simulink model "mpc_psm"  (R2026b)
settings: Solver=ode23tb  StopTime=param.sim.simlength  FixedStep=param.glb_time.tc  MaxStep=param.glb_time.tc
values from neighbouring files (symbols this model uses):
  param = struct()    [init_model.m]
undefined symbols (not defined in the file or in its folder): tc
libraries: fl_lib x28, nesl_utility x13, cstblocks_lti x6, lithium_ion_battery x1, dclink_with_center_tap x1, ideal_bridges_lib x1, dead_time_generator_cmos_simulink x1, single_phase_pwm_modulator x1, threephase_inductor_lib x1, simple_flexible_shaft x1, permanent_magnet_synchronous_machine x1
(part 2 of 3)

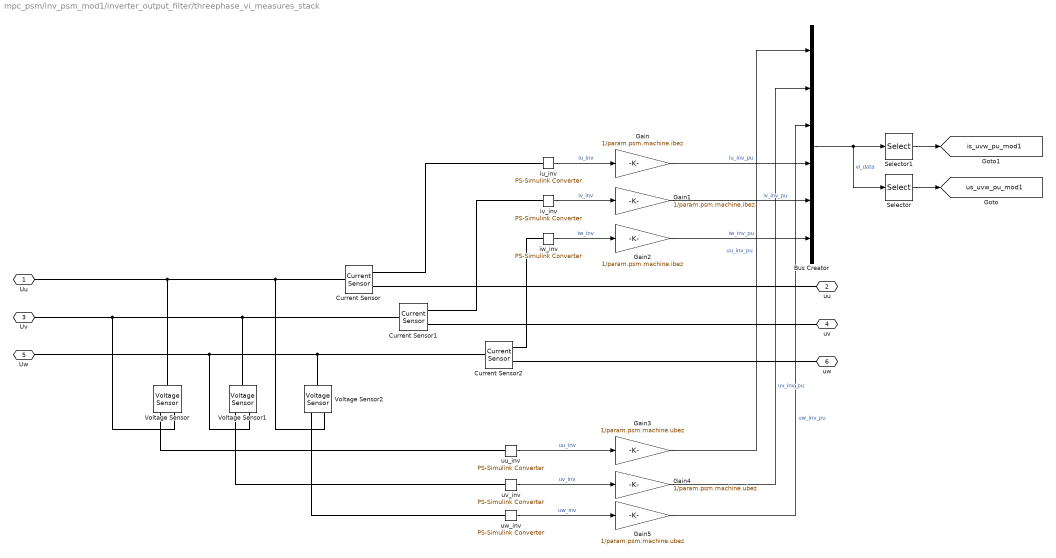
== system mpc_psm/inv_psm_mod1/inverter_output_filter/threephase_vi_measures_stack ==
  Bus Creator : BusCreator  Inputs=6
  Current Sensor : fl_lib/Electrical/Electrical Sensors/Current Sensor
  Current Sensor1 : fl_lib/Electrical/Electrical Sensors/Current Sensor
  Current Sensor2 : fl_lib/Electrical/Electrical Sensors/Current Sensor
  Gain : Gain  Gain=1/param.psm.machine.ibez
  Gain1 : Gain  Gain=1/param.psm.machine.ibez
  Gain2 : Gain  Gain=1/param.psm.machine.ibez
  Gain3 : Gain  Gain=1/param.psm.machine.ubez
  Gain4 : Gain  Gain=1/param.psm.machine.ubez
  Gain5 : Gain  Gain=1/param.psm.machine.ubez
  Selector : Selector  InputPortWidth=6  IndexOptions=Index vector (dialog)  Indices=[1 2 3]  OutputSizes=1  RuntimeRangeChecks=off
  Selector1 : Selector  InputPortWidth=6  IndexOptions=Index vector (dialog)  Indices=[4 5 6]  OutputSizes=1  RuntimeRangeChecks=off
  Voltage Sensor : fl_lib/Electrical/Electrical Sensors/Voltage Sensor
  Voltage Sensor1 : fl_lib/Electrical/Electrical Sensors/Voltage Sensor
  Voltage Sensor2 : fl_lib/Electrical/Electrical Sensors/Voltage Sensor
  iu_inv : nesl_utility/PS-Simulink Converter  PhysicalDomain=network_engine_domain  SubClassName=ps_output  LeftPortType=input  RightPortType=output  PseudoPeriodic=off  Frequencies=[]  VectorFormat=1-D array  Unit=A  AffineConversion=off
  iv_inv : nesl_utility/PS-Simulink Converter  PhysicalDomain=network_engine_domain  SubClassName=ps_output  LeftPortType=input  RightPortType=output  PseudoPeriodic=off  Frequencies=[]  VectorFormat=1-D array  Unit=A  AffineConversion=off
  iw_inv : nesl_utility/PS-Simulink Converter  PhysicalDomain=network_engine_domain  SubClassName=ps_output  LeftPortType=input  RightPortType=output  PseudoPeriodic=off  Frequencies=[]  VectorFormat=1-D array  Unit=A  AffineConversion=off
  uu_inv : nesl_utility/PS-Simulink Converter  PhysicalDomain=network_engine_domain  SubClassName=ps_output  LeftPortType=input  RightPortType=output  PseudoPeriodic=off  Frequencies=[]  VectorFormat=1-D array  Unit=V  AffineConversion=off
  uv_inv : nesl_utility/PS-Simulink Converter  PhysicalDomain=network_engine_domain  SubClassName=ps_output  LeftPortType=input  RightPortType=output  PseudoPeriodic=off  Frequencies=[]  VectorFormat=1-D array  Unit=V  AffineConversion=off
  uw_inv : nesl_utility/PS-Simulink Converter  PhysicalDomain=network_engine_domain  SubClassName=ps_output  LeftPortType=input  RightPortType=output  PseudoPeriodic=off  Frequencies=[]  VectorFormat=1-D array  Unit=V  AffineConversion=off
  Uu : PMIOPort  Side=Left
  uu : PMIOPort  Port=2  Side=Right
  Uv : PMIOPort  Port=3  Side=Left
  uv : PMIOPort  Port=4  Side=Right
  Uw : PMIOPort  Port=5  Side=Left
  uw : PMIOPort  Port=6  Side=Right
  tag scope: is_uvw_pu_mod1=global, us_uvw_pu_mod1=global
  wires:
  Bus Creator/1 -> Selector/1, Selector1/1  "vi_data"
  Selector/1 -> [us_uvw_pu_mod1]
  iv_inv/1 -> Gain1/1  "iv_inv"
  iu_inv/1 -> Gain/1  "iu_inv"
  iw_inv/1 -> Gain2/1  "iw_inv"
  uu_inv/1 -> Gain3/1  "uu_inv"
  uv_inv/1 -> Gain4/1  "uv_inv"
  uw_inv/1 -> Gain5/1  "uw_inv"
  Selector1/1 -> [is_uvw_pu_mod1]
  Gain/1 -> Bus Creator/4  "iu_inv_pu"
  Gain1/1 -> Bus Creator/5  "iv_inv_pu"
  Gain2/1 -> Bus Creator/6  "iw_inv_pu"
  Gain3/1 -> Bus Creator/1  "uu_inv_pu"
  Gain4/1 -> Bus Creator/2  "uv_inv_pu"
  Gain5/1 -> Bus Creator/3  "uw_inv_pu"
  connections:
  Current Sensor1/LConn1 -- Voltage Sensor1/LConn1 -- Voltage Sensor/RConn2 -- Uv/RConn1
  Voltage Sensor/RConn1 -- uu_inv/LConn1
  Current Sensor/RConn2 -- uu/RConn1
  Voltage Sensor1/RConn1 -- uv_inv/LConn1
  Voltage Sensor2/LConn1 -- Current Sensor2/LConn1 -- Voltage Sensor1/RConn2 -- Uw/RConn1
  Current Sensor/LConn1 -- Voltage Sensor2/RConn2 -- Uu/RConn1 -- Voltage Sensor/LConn1
  Current Sensor1/RConn2 -- uv/RConn1
  Voltage Sensor2/RConn1 -- uw_inv/LConn1
  iv_inv/LConn1 -- Current Sensor1/RConn1
  iu_inv/LConn1 -- Current Sensor/RConn1
  iw_inv/LConn1 -- Current Sensor2/RConn1
  Current Sensor2/RConn2 -- uw/RConn1

== system mpc_psm/inv_psm_mod1/inverter/inverter/timer ==
  time_source : Inport
  Constant1 : Constant  Value=double_sampling
  Constant2 : Constant  Value=0
  Constant8 : Constant  Value=tc
  Constant9 : Constant  Value=f
  MATLAB Function : MATLAB Function  TreatAsAtomicUnit=on  SystemSampleTime=tc
  MATLAB Function1 : single_phase_pwm_modulator/Single phase two level PWM generator with global TRGO/MATLAB Function1  SystemSampleTime=tc  VariantActivationTime=update diagram  EmptyChoice=off  PassThrough=off  PassThroughVariantControl=(default)  EmptyChoiceVariantControl=(default)  AllowFlexibleInterface=on  Latency=0  AutoFrameSizeCalculation=off
  period : Constant  Value=1/f
  TRGO : Outport
  wires:
  Constant1/1 -> MATLAB Function1/4
  time_source/1 -> MATLAB Function/1(t)
  Constant9/1 -> MATLAB Function1/2
  Constant8/1 -> MATLAB Function1/1
  MATLAB Function1/1 -> TRGO/1
  MATLAB Function/1(y) -> MATLAB Function1/3
  Constant2/1 -> MATLAB Function/2(phase)
  period/1 -> MATLAB Function/3(period)

== system mpc_psm/inv_psm_mod1/inverter_ctrl/inverter_control/Speed control ==
  rotor speed : Inport
  rotor speed ref : Inport  Port=2
  1/Ti : Gain  Gain=param.psm.ctrl.kp_w  SaturateOnIntegerOverflow=on  OutDataTypeStr=Inherit: Same as input  ParamDataTypeStr=Inherit: Same as input
  Saturation : Saturate  UpperLimit=param.psm.ctrl.iq_lim  LowerLimit=-param.psm.ctrl.iq_lim
  Sum1 : Sum  Inputs=+++  SaturateOnIntegerOverflow=on
  Sum2 : Sum  Inputs=-+  SaturateOnIntegerOverflow=on
  Sum3 : Sum  Inputs=-+  SaturateOnIntegerOverflow=on
  Unit Delay4 : UnitDelay  SampleTime=-1
  kp : Gain  Gain=param.psm.ctrl.ki_w*param.glb_time.ts_inv  SaturateOnIntegerOverflow=on  OutDataTypeStr=Inherit: Same as input  ParamDataTypeStr=Inherit: Same as input
  torque_ref : Outport
  wires:
  1/Ti/1 -> Sum1/1, Sum3/1
  kp/1 -> Sum1/2
  Sum3/1 -> Unit Delay4/1
  Unit Delay4/1 -> Sum1/3
  rotor speed ref/1 -> Sum2/2
  rotor speed/1 -> Sum2/1
  Sum2/1 -> kp/1, 1/Ti/1
  Sum1/1 -> Saturation/1
  Saturation/1 -> Sum3/2, torque_ref/1

== system mpc_psm/inv_psm_mod1/inverter_ctrl/inverter_control/encoder-sensorless-switch ==
  Constant : Constant  Value=param.psm.ctrl.omega_th
  MATLAB Function : MATLAB Function  TreatAsAtomicUnit=on
  Variant Source1 : VariantSource  VariantControls={param.psm.mode.use_psm_encoder == 1, param.psm.mode.use_psm_encoder == 0}
  Variant Source2 : VariantSource  VariantControls={param.psm.mode.use_psm_encoder == 1, param.psm.mode.use_psm_encoder == 0}
  double_integrator_observer : Subsystem
  omega_pu_psm/hat1 : Scope  NumInputPorts=2
      settings: ActiveDisplayYMinimum=0.7763345893279654  ActiveDisplayYMaximum=1.2909010705406665  DataLoggingVariableName=ScopeData13
  theta_elec_psm/hat : Scope  NumInputPorts=2
      settings: ActiveDisplayYMinimum=-1  ActiveDisplayYMaximum=1  DataLoggingVariableName=ScopeData12
  tag scope: motor_phase_ctrl_mod1=scoped, motor_speed_pu_ctrl_mod1=scoped
  wires:
  Variant Source1/1 -> [motor_speed_pu_ctrl_mod1]
  Variant Source2/1 -> [motor_phase_ctrl_mod1]
  [phase_hat_mod1] -> theta_elec_psm/hat/1  "theta_hat_mod1"
  [omega_hat_pu_mod1] -> omega_pu_psm/hat1/1  "omega_hat_pu_mod1"
  [phased_psm] -> double_integrator_observer/1(phase_psm)
  double_integrator_observer/1(omega_pu_psm_hat) -> MATLAB Function/1(omega_psm), Variant Source1/1, omega_pu_psm/hat1/2  "omega_pu_psm_hat"
  double_integrator_observer/2(phase_psm_hat) -> theta_elec_psm/hat/2, Variant Source2/1, MATLAB Function/2(phase_psm)  "theta_psm_hat"
  MATLAB Function/1(omega_ctrl) -> Variant Source1/2
  MATLAB Function/2(phase_ctrl) -> Variant Source2/2
  [omega_hat_pu_mod1] -> MATLAB Function/3(omega_obs)  "omega_hat_pu_mod1"
  [phase_hat_mod1] -> MATLAB Function/4(phase_obs)  "theta_hat_mod1"
  Constant/1 -> MATLAB Function/5(omega_th)

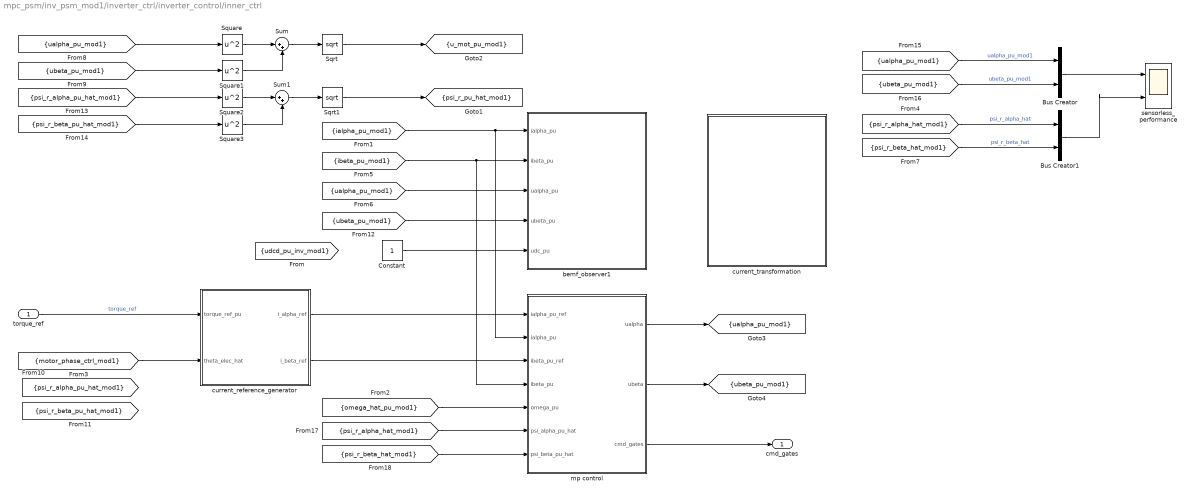
== system mpc_psm/inv_psm_mod1/inverter_ctrl/inverter_control/inner_ctrl ==
  torque_ref : Inport
  Bus Creator : BusCreator  Inputs=2
  Bus Creator1 : BusCreator  Inputs=2
  Constant : Constant
  Sqrt : Sqrt
  Sqrt1 : Sqrt
  Square{,1..3} (4 alike) : Math  Operator=square
  Sum : Sum  Inputs=|++
  Sum1 : Sum  Inputs=|++
  bemf_observer1 : Subsystem
  current_reference_generator : Subsystem
  current_transformation : Subsystem
  mp control : Subsystem
  sensorless_performance : Scope  NumInputPorts=2
      settings: ActiveDisplayYMinimum=-1.21322413533926  ActiveDisplayYMaximum=1.2041211351752281  DataLoggingVariableName=ScopeData5
  cmd_gates : Outport  VectorParamsAs1DForOutWhenUnconnected=off
  tag scope: psi_r_pu_hat_mod1=scoped, u_mot_pu_mod1=scoped, ualpha_pu_mod1=scoped, ubeta_pu_mod1=scoped
  wires:
  torque_ref/1 -> current_reference_generator/1(torque_ref_pu)  "torque_ref"
  [ibeta_pu_mod1] -> bemf_observer1/2(ibeta_pu), mp control/4(ibeta_pu)
  [ialpha_pu_mod1] -> bemf_observer1/1(ialpha_pu), mp control/2(ialpha_pu)
  [ualpha_pu_mod1] -> bemf_observer1/3(ualpha_pu)
  [ubeta_pu_mod1] -> bemf_observer1/4(ubeta_pu)
  Constant/1 -> bemf_observer1/5(udc_pu)
  [motor_phase_ctrl_mod1] -> current_reference_generator/2(theta_elec_hat)
  mp control/1(ualpha) -> [ualpha_pu_mod1]
  mp control/2(ubeta) -> [ubeta_pu_mod1]
  current_reference_generator/1(i_alpha_ref) -> mp control/1(ialpha_pu_ref)
  current_reference_generator/2(i_beta_ref) -> mp control/3(ibeta_pu_ref)
  [omega_hat_pu_mod1] -> mp control/5(omega_pu)
  [psi_r_alpha_hat_mod1] -> mp control/6(psi_alpha_pu_hat)
  [psi_r_beta_hat_mod1] -> mp control/7(psi_beta_pu_hat)
  mp control/3(cmd_gates) -> cmd_gates/1
  [ualpha_pu_mod1] -> Square/1
  [ubeta_pu_mod1] -> Square1/1
  Square/1 -> Sum/1
  Square1/1 -> Sum/2
  Sum/1 -> Sqrt/1
  Sqrt/1 -> [u_mot_pu_mod1]
  Sqrt1/1 -> [psi_r_pu_hat_mod1]
  Sum1/1 -> Sqrt1/1
  Square3/1 -> Sum1/2
  Square2/1 -> Sum1/1
  [psi_r_beta_pu_hat_mod1] -> Square3/1
  [psi_r_alpha_pu_hat_mod1] -> Square2/1
  [ualpha_pu_mod1] -> Bus Creator/1  "ualpha_pu_mod1"
  [ubeta_pu_mod1] -> Bus Creator/2  "ubeta_pu_mod1"
  [psi_r_beta_hat_mod1] -> Bus Creator1/2  "psi_r_beta_hat"
  [psi_r_alpha_hat_mod1] -> Bus Creator1/1  "psi_r_alpha_hat"
  Bus Creator/1 -> sensorless_performance/1
  Bus Creator1/1 -> sensorless_performance/2

== system mpc_psm/inv_psm_mod1/inverter_ctrl/inverter_control/is inv quantizzation and one step delay ==
  is_abc_pu : Inport
  Demux : Demux  Outputs=3
  Mux : Mux  Inputs=3
  is inv quantizzation and one step delay : Subsystem
  isd_abc_pu : Outport
  wires:
  is inv quantizzation and one step delay/2(isd_v_pu) -> Mux/2
  is_abc_pu/1 -> Demux/1
  is inv quantizzation and one step delay/3(isd_w_pu) -> Mux/3
  is inv quantizzation and one step delay/1(isd_u_pu) -> Mux/1
  Demux/1 -> is inv quantizzation and one step delay/1(is_u_pu)
  Mux/1 -> isd_abc_pu/1
  Demux/3 -> is inv quantizzation and one step delay/3(is_w_pu)
  Demux/2 -> is inv quantizzation and one step delay/2(is_v_pu)

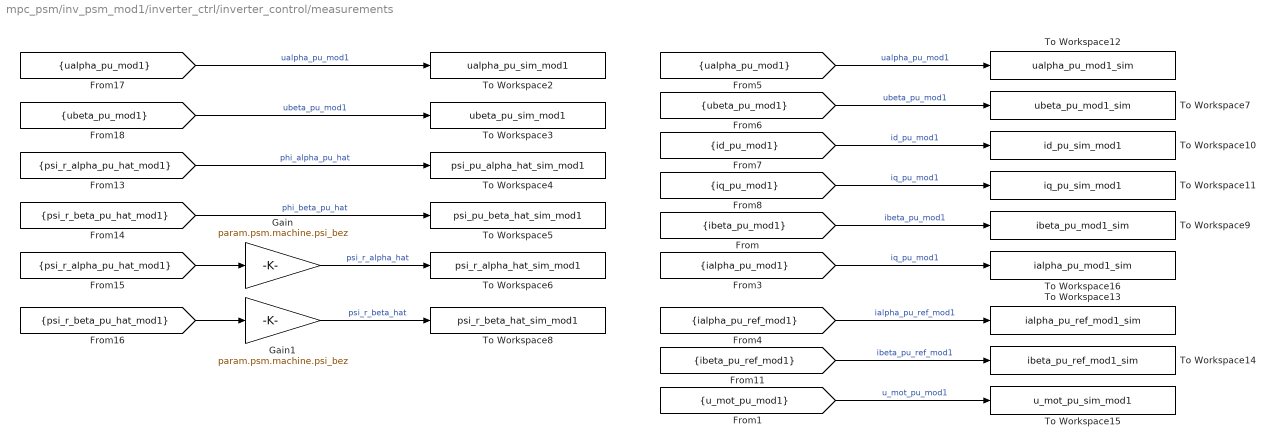
== system mpc_psm/inv_psm_mod1/inverter_ctrl/inverter_control/measurements ==
  Gain : Gain  Gain=param.psm.machine.psi_bez
  Gain1 : Gain  Gain=param.psm.machine.psi_bez
  To Workspace10 : ToWorkspace  VariableName=id_pu_sim_mod1  SampleTime=-1
      settings: MaxDataPoints=param.glb_time.Ns_inv
  To Workspace11 : ToWorkspace  VariableName=iq_pu_sim_mod1  SampleTime=-1
      settings: MaxDataPoints=param.glb_time.Ns_inv
  To Workspace12 : ToWorkspace  VariableName=ualpha_pu_mod1_sim  SampleTime=-1
      settings: MaxDataPoints=param.glb_time.Ns_inv
  To Workspace13 : ToWorkspace  VariableName=ialpha_pu_ref_mod1_sim  SampleTime=-1
      settings: MaxDataPoints=param.glb_time.Ns_inv
  To Workspace14 : ToWorkspace  VariableName=ibeta_pu_ref_mod1_sim  SampleTime=-1
      settings: MaxDataPoints=param.glb_time.Ns_inv
  To Workspace15 : ToWorkspace  VariableName=u_mot_pu_sim_mod1  SampleTime=-1
      settings: MaxDataPoints=param.glb_time.Ns_inv
  To Workspace16 : ToWorkspace  VariableName=ialpha_pu_mod1_sim  SampleTime=-1
      settings: MaxDataPoints=param.glb_time.Ns_inv
  To Workspace2 : ToWorkspace  VariableName=ualpha_pu_sim_mod1  SampleTime=-1
      settings: MaxDataPoints=param.glb_time.Ns_inv
  To Workspace3 : ToWorkspace  VariableName=ubeta_pu_sim_mod1  SampleTime=-1
      settings: MaxDataPoints=param.glb_time.Ns_inv
  To Workspace4 : ToWorkspace  VariableName=psi_pu_alpha_hat_sim_mod1  SampleTime=-1
      settings: MaxDataPoints=param.glb_time.Ns_inv
  To Workspace5 : ToWorkspace  VariableName=psi_pu_beta_hat_sim_mod1  SampleTime=-1
      settings: MaxDataPoints=param.glb_time.Ns_inv
  To Workspace6 : ToWorkspace  VariableName=psi_r_alpha_hat_sim_mod1  SampleTime=-1
      settings: MaxDataPoints=param.glb_time.Ns_inv
  To Workspace7 : ToWorkspace  VariableName=ubeta_pu_mod1_sim  SampleTime=-1
      settings: MaxDataPoints=param.glb_time.Ns_inv
  To Workspace8 : ToWorkspace  VariableName=psi_r_beta_hat_sim_mod1  SampleTime=-1
      settings: MaxDataPoints=param.glb_time.Ns_inv
  To Workspace9 : ToWorkspace  VariableName=ibeta_pu_mod1_sim  SampleTime=-1
      settings: MaxDataPoints=param.glb_time.Ns_inv
  wires:
  [psi_r_alpha_pu_hat_mod1] -> Gain/1
  [ualpha_pu_mod1] -> To Workspace2/1  "ualpha_pu_mod1"
  Gain/1 -> To Workspace6/1  "psi_r_alpha_hat"
  [psi_r_alpha_pu_hat_mod1] -> To Workspace4/1  "phi_alpha_pu_hat"
  [ubeta_pu_mod1] -> To Workspace3/1  "ubeta_pu_mod1"
  [psi_r_beta_pu_hat_mod1] -> To Workspace5/1  "phi_beta_pu_hat"
  Gain1/1 -> To Workspace8/1  "psi_r_beta_hat"
  [psi_r_beta_pu_hat_mod1] -> Gain1/1
  [u_mot_pu_mod1] -> To Workspace15/1  "u_mot_pu_mod1"
  [ialpha_pu_ref_mod1] -> To Workspace13/1  "ialpha_pu_ref_mod1"
  [ubeta_pu_mod1] -> To Workspace7/1  "ubeta_pu_mod1"
  [ualpha_pu_mod1] -> To Workspace12/1  "ualpha_pu_mod1"
  [iq_pu_mod1] -> To Workspace11/1  "iq_pu_mod1"
  [id_pu_mod1] -> To Workspace10/1  "id_pu_mod1"
  [ibeta_pu_ref_mod1] -> To Workspace14/1  "ibeta_pu_ref_mod1"
  [ibeta_pu_mod1] -> To Workspace9/1  "ibeta_pu_mod1"
  [ialpha_pu_mod1] -> To Workspace16/1  "iq_pu_mod1"

== system mpc_psm/inv_psm_mod1/inverter_ctrl/inverter_control/omega_acquisition ==
  omega_psm : Inport
  Gain : Gain  Gain=1/param.psm.machine.omega_bez
  Quantizer : Quantizer  QuantizationInterval=param.meas.adc_quantization
  Unit Delay : UnitDelay  SampleTime=-1
  Zero-Order Hold : ZeroOrderHold  SampleTime=-1
  omega_pu_psm : Outport
  wires:
  Quantizer/1 -> Unit Delay/1
  omega_psm/1 -> Gain/1
  Unit Delay/1 -> omega_pu_psm/1
  Zero-Order Hold/1 -> Quantizer/1
  Gain/1 -> Zero-Order Hold/1

== system mpc_psm/inv_psm_mod1/inverter_ctrl/inverter_control/omega_pu ==
  Abs : Abs  SaturateOnIntegerOverflow=off
  flt : Subsystem
  abs(omega_pu) : Outport
  omega_pu : Outport  Port=2
  wires:
  Abs/1 -> flt/1(input)
  [motor_speed_pu_ctrl_mod1] -> Abs/1, omega_pu/1
  flt/1(output) -> abs(omega_pu)/1

== system mpc_psm/inv_psm_mod1/inverter_ctrl/inverter_control/phase_acquisition ==
  phase_psm : Inport
  Quantizer : Quantizer  QuantizationInterval=param.meas.adc_quantization
  Unit Delay : UnitDelay  SampleTime=-1
  Zero-Order Hold : ZeroOrderHold  SampleTime=-1
  phased_psm : Outport
  wires:
  Zero-Order Hold/1 -> Quantizer/1
  Unit Delay/1 -> phased_psm/1
  phase_psm/1 -> Zero-Order Hold/1
  Quantizer/1 -> Unit Delay/1

== system mpc_psm/inv_psm_mod1/inverter_ctrl/inverter_control/phase_compensation_1 ==
  local_time : Inport
  master_time : Inport  Port=2
  Zero-Order Hold : ZeroOrderHold  SampleTime=-1
  Zero-Order Hold1 : ZeroOrderHold  SampleTime=-1
  alignment_ctrl : Subsystem
  y : Outport
  wires:
  local_time/1 -> Zero-Order Hold/1
  master_time/1 -> Zero-Order Hold1/1
  alignment_ctrl/1(dp) -> y/1
  Zero-Order Hold/1 -> alignment_ctrl/1(local_time)
  Zero-Order Hold1/1 -> alignment_ctrl/2(master_time)

== system mpc_psm/inv_psm_mod1/inverter_ctrl/inverter_control/speed_reference_generator ==
  Step : Step  Time=param.psm.mode.time_start_motor_control  FinalValue=param.load.omega_m_sim/param.psm.machine.omega_m_bez
  Step1 : Step  Commented=on  Time=param.sim.simlength/2  FinalValue=-2*param.load.omega_m_sim/param.psm.machine.omega_m_bez
  Sum : Sum  Inputs=|++
  flt : Subsystem
  omega_ref_pu : Outport
  tag scope: omega_ref_pu_mod1=global
  wires:
  Step/1 -> Sum/1
  Step1/1 -> Sum/2
  Sum/1 -> flt/1(input)
  flt/1(output) -> [omega_ref_pu_mod1], omega_ref_pu/1

== system mpc_psm/inv_psm_mod1/inverter_ctrl/inverter_control/torque_reference ==
  rotor speed : Inport
  1-D Lookup Table : Lookup_n-D  NumberOfTableDimensions=1  BreakpointsForDimension1=param.load.rpm_base  Table=param.load.torque_base  InternalRulePriority=Speed  RndMeth=Simplest
  Gain : Gain  Gain=param.load.torque_overload_factor
  Gain1 : Gain  Gain=1/param.psm.machine.tau_bez
  Gain2 : Gain  Gain=param.psm.machine.rpm_nom
  Gain3 : Gain  Gain=-1
  Saturation : Saturate  UpperLimit=0  LowerLimit=-inf
  torque_ref : Outport
  wires:
  rotor speed/1 -> Gain2/1
  Gain/1 -> Saturation/1
  Saturation/1 -> torque_ref/1
  Gain1/1 -> Gain3/1
  1-D Lookup Table/1 -> Gain1/1
  Gain2/1 -> 1-D Lookup Table/1
  Gain3/1 -> Gain/1

== system mpc_psm/inv_psm_mod1/inverter_ctrl/inverter_control/udc_acquisition ==
  udc_pu : Inport
  Quantizer : Quantizer  QuantizationInterval=param.meas.adc_quantization
  Unit Delay : UnitDelay  SampleTime=-1
  Zero-Order Hold : ZeroOrderHold  SampleTime=-1
  udcd_pu : Outport
  wires:
  Quantizer/1 -> Unit Delay/1
  udc_pu/1 -> Zero-Order Hold/1
  Unit Delay/1 -> udcd_pu/1
  Zero-Order Hold/1 -> Quantizer/1

== system mpc_psm/inv_psm_mod1/inverter_ctrl/inverter_control/encoder-sensorless-switch/double_integrator_observer ==
  phase_psm : Inport
  Dead Zone : DeadZone  LowerValue=-0.01  UpperValue=0.01
  Gain : Gain  Gain=param.psm.ctrl.di_obs.komega
  Gain1 : Gain  Gain=param.psm.ctrl.di_obs.ktheta
  Gain2 : Gain  Gain=param.psm.ctrl.omega_base
  Gain3 : Gain  Gain=1/param.psm.ctrl.omega_base
  Gain4 : Gain  Gain=param.glb_time.ts_inv
  Gain5 : Gain  Gain=param.glb_time.ts_inv
  Gain6 : Gain  Gain=param.glb_time.ts_inv
  Sum : Sum  Inputs=-+|
  Sum1 : Sum  Inputs=|++
  Sum2 : Sum  Inputs=|++
  Sum8 : Sum  Inputs=++|
  Unit Delay1 : UnitDelay  InitialCondition=pi  SampleTime=-1
  Unit Delay2 : UnitDelay  SampleTime=-1
  bounder1 : MATLAB Function  TreatAsAtomicUnit=on
  bounder2 : MATLAB Function  TreatAsAtomicUnit=on
  omega_pu_psm_hat : Outport  VectorParamsAs1DForOutWhenUnconnected=off
  phase_psm_hat : Outport  Port=2  VectorParamsAs1DForOutWhenUnconnected=off
  wires:
  Gain1/1 -> Gain6/1
  phase_psm/1 -> Sum/2
  Sum8/1 -> Unit Delay1/1
  Unit Delay1/1 -> bounder2/1(u)
  Sum1/1 -> Unit Delay2/1
  Gain/1 -> Gain4/1
  Unit Delay2/1 -> omega_pu_psm_hat/1, Sum1/2, Gain5/1
  Sum2/1 -> Sum8/2
  bounder2/1(y) -> Sum2/2, phase_psm_hat/1, Sum/1  "phase_hat"
  bounder1/1(y) -> Gain1/1, Gain/1
  Gain2/1 -> Sum8/1
  Gain3/1 -> Sum1/1
  Gain5/1 -> Gain2/1
  Sum/1 -> bounder1/1(u)
  Gain4/1 -> Gain3/1
  Gain6/1 -> Sum2/1

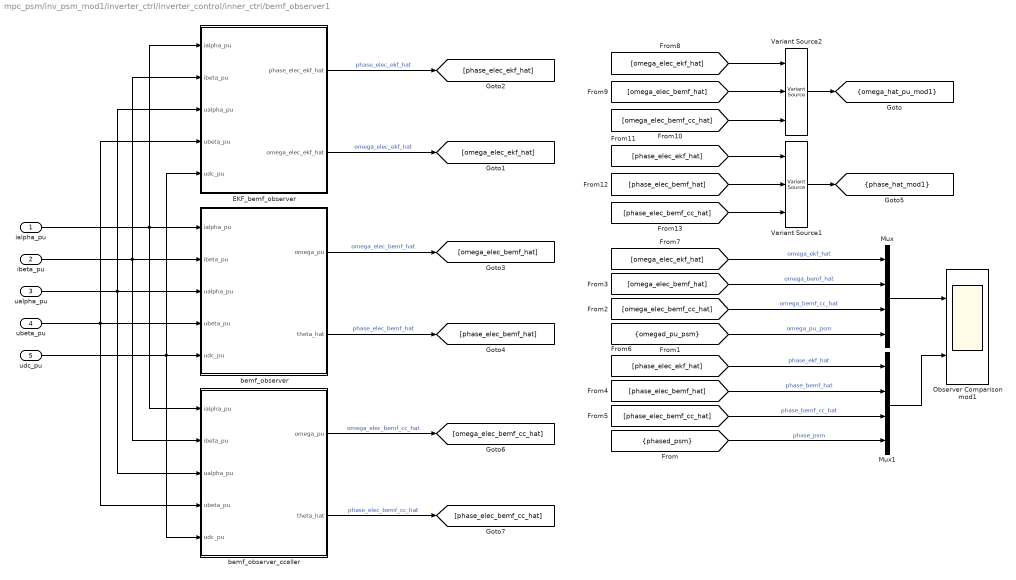
== system mpc_psm/inv_psm_mod1/inverter_ctrl/inverter_control/inner_ctrl/bemf_observer1 ==
  ialpha_pu : Inport
  ibeta_pu : Inport  Port=2
  ualpha_pu : Inport  Port=3
  ubeta_pu : Inport  Port=4
  udc_pu : Inport  Port=5
  EKF_bemf_observer : Subsystem
  Mux : Mux
  Mux1 : Mux
  Observer Comparison mod1 : Scope  NumInputPorts=2
      settings: ActiveDisplayYMinimum=-1.7949249844307968  ActiveDisplayYMaximum=1.3113178143582995
  Variant Source1 : VariantSource  VariantControls={param.psm.impl.use_ekf_bemf_module_1 == 1, param.psm.impl.use_observer_from_simulink_module_1 == 1, param.psm.impl.use_observer_from_ccaller_module_1 == 1}
  Variant Source2 : VariantSource  VariantControls={param.psm.impl.use_ekf_bemf_module_1 == 1, param.psm.impl.use_observer_from_simulink_module_1 == 1, param.psm.impl.use_observer_from_ccaller_module_1 == 1}
  bemf_observer : Subsystem
  bemf_observer_ccaller : Subsystem
  tag scope: omega_hat_pu_mod1=scoped, phase_hat_mod1=scoped
  wires:
  ialpha_pu/1 -> EKF_bemf_observer/1(ialpha_pu), bemf_observer_ccaller/1(ialpha_pu), bemf_observer/1(ialpha_pu)
  ibeta_pu/1 -> EKF_bemf_observer/2(ibeta_pu), bemf_observer_ccaller/2(ibeta_pu), bemf_observer/2(ibeta_pu)
  Mux/1 -> Observer Comparison mod1/1
  Mux1/1 -> Observer Comparison mod1/2
  ualpha_pu/1 -> EKF_bemf_observer/3(ualpha_pu), bemf_observer_ccaller/3(ualpha_pu), bemf_observer/3(ualpha_pu)
  ubeta_pu/1 -> EKF_bemf_observer/4(ubeta_pu), bemf_observer_ccaller/4(ubeta_pu), bemf_observer/4(ubeta_pu)
  Variant Source1/1 -> [phase_hat_mod1]
  Variant Source2/1 -> [omega_hat_pu_mod1]
  udc_pu/1 -> EKF_bemf_observer/5(udc_pu), bemf_observer_ccaller/5(udc_pu), bemf_observer/5(udc_pu)
  [omegad_pu_psm] -> Mux/4  "omega_pu_psm"
  [phased_psm] -> Mux1/4  "phase_psm"
  EKF_bemf_observer/2(omega_elec_ekf_hat) -> [omega_elec_ekf_hat]  "omega_elec_ekf_hat"
  EKF_bemf_observer/1(phase_elec_ekf_hat) -> [phase_elec_ekf_hat]  "phase_elec_ekf_hat"
  bemf_observer/1(omega_pu) -> [omega_elec_bemf_hat]  "omega_elec_bemf_hat"
  bemf_observer/2(theta_hat) -> [phase_elec_bemf_hat]  "phase_elec_bemf_hat"
  bemf_observer_ccaller/2(theta_hat) -> [phase_elec_bemf_cc_hat]  "phase_elec_bemf_cc_hat"
  bemf_observer_ccaller/1(omega_pu) -> [omega_elec_bemf_cc_hat]  "omega_elec_bemf_cc_hat"
  [phase_elec_bemf_cc_hat] -> Mux1/3  "phase_bemf_cc_hat"
  [omega_elec_bemf_cc_hat] -> Mux/3  "omega_bemf_cc_hat"
  [omega_elec_bemf_hat] -> Mux/2  "omega_bemf_hat"
  [phase_elec_bemf_hat] -> Mux1/2  "phase_bemf_hat"
  [phase_elec_ekf_hat] -> Mux1/1  "phase_ekf_hat"
  [omega_elec_ekf_hat] -> Mux/1  "omega_ekf_hat"
  [omega_elec_ekf_hat] -> Variant Source2/1
  [omega_elec_bemf_hat] -> Variant Source2/2
  [omega_elec_bemf_cc_hat] -> Variant Source2/3
  [phase_elec_ekf_hat] -> Variant Source1/1
  [phase_elec_bemf_hat] -> Variant Source1/2
  [phase_elec_bemf_cc_hat] -> Variant Source1/3

== system mpc_psm/inv_psm_mod1/inverter_ctrl/inverter_control/inner_ctrl/current_reference_generator ==
  torque_ref_pu : Inport
  theta_elec_hat : Inport  Port=2
  Gain5 : Gain  Gain=-1
  Product : Product
  Product1 : Product
  Trigonometric Function1 : Trigonometry
  Trigonometric Function2 : Trigonometry  Operator=cos
  i_alpha_ref : Outport
  i_beta_ref : Outport  Port=2
  tag scope: ialpha_pu_ref_mod1=scoped, ibeta_pu_ref_mod1=scoped
  wires:
  Trigonometric Function1/1 -> Product/2
  Product1/1 -> [ibeta_pu_ref_mod1], i_beta_ref/1
  Trigonometric Function2/1 -> Product1/2
  Product/1 -> Gain5/1
  Gain5/1 -> [ialpha_pu_ref_mod1], i_alpha_ref/1
  torque_ref_pu/1 -> Product/1, Product1/1
  theta_elec_hat/1 -> Trigonometric Function1/1, Trigonometric Function2/1  "theta_electrical"

== system mpc_psm/inv_psm_mod1/inverter_ctrl/inverter_control/inner_ctrl/current_transformation ==
  Demux : Demux  Outputs=3
  alphabeta2dq : MATLAB Function  TreatAsAtomicUnit=on
  uvw2alphabeta : MATLAB Function  TreatAsAtomicUnit=on
  tag scope: ialpha_pu_mod1=scoped, ibeta_pu_mod1=scoped, id_pu_mod1=scoped, iq_pu_mod1=scoped
  wires:
  alphabeta2dq/2(q) -> [iq_pu_mod1]  "iq_pu"
  alphabeta2dq/1(d) -> [id_pu_mod1]  "id_pu"
  uvw2alphabeta/2(beta) -> alphabeta2dq/2(beta), [ibeta_pu_mod1]  "ibeta_pu"
  uvw2alphabeta/1(alpha) -> [ialpha_pu_mod1], alphabeta2dq/1(alpha)  "ialpha_pu"
  [motor_phase_ctrl_mod1] -> alphabeta2dq/3(gamma)
  Demux/3 -> uvw2alphabeta/3(w)  "iw"
  Demux/2 -> uvw2alphabeta/2(v)  "iv"
  Demux/1 -> uvw2alphabeta/1(u)  "iu"
  [isd_uvw_inv_mod1] -> Demux/1

== system mpc_psm/inv_psm_mod1/inverter_ctrl/inverter_control/inner_ctrl/mp control ==
  ialpha_pu_ref : Inport
  ialpha_pu : Inport  Port=2
  ibeta_pu_ref : Inport  Port=3
  ibeta_pu : Inport  Port=4
  omega_pu : Inport  Port=5
  psi_alpha_pu_hat : Inport  Port=6
  psi_beta_pu_hat : Inport  Port=7
  Bus Creator : BusCreator  Inputs=6
  Bus Creator1 : BusCreator  Inputs=2
  Bus Creator2 : BusCreator  Inputs=2
  Constant1 : Constant  Value=param.psm.ctrl.mpc.u_scale
  Constant2 : Constant  Value=param.psm.ctrl.mpc.L_norm
  Constant3 : Constant  Value=param.psm.machine.omega_bez
  Constant4 : Constant  Value=param.psm.ctrl.mpc.R_norm
  Constant5 : Constant  Value=param.psm.ctrl.mpc.k_kalman
  Constant6 : Constant  Value=param.psm.ctrl.mpc.k_sw
  Constant7 : Constant  Value=param.glb_time.ts_inv
  Gain1 : Gain  Gain=1
  Gain7 : Gain  Gain=1
  Unit Delay : UnitDelay  SampleTime=-1
  Unit Delay1 : UnitDelay  SampleTime=-1
  ialpha/beta_tracking : Scope  NumInputPorts=2
      settings: ActiveDisplayYMinimum=-0.330322265625  ActiveDisplayYMaximum=0.360595703125  DataLoggingVariableName=ScopeData2
  mpc_pu_d : MATLAB Function  TreatAsAtomicUnit=on
  ualpha : Outport
  ubeta : Outport  Port=2
  cmd_gates : Outport  Port=3
  wires:
  ialpha_pu_ref/1 -> Bus Creator1/1, mpc_pu_d/2(ialpha_ref)  "ialpha_pu_ref"
  ibeta_pu_ref/1 -> Bus Creator2/1, mpc_pu_d/3(ibeta_ref)  "ibeta_pu_ref"
  ialpha_pu/1 -> Bus Creator1/2, mpc_pu_d/4(ialpha)  "ialpha_pu"
  ibeta_pu/1 -> mpc_pu_d/5(ibeta), Bus Creator2/2  "ibeta_pu"
  omega_pu/1 -> mpc_pu_d/6(omega_hat)  "omega_hat"
  psi_alpha_pu_hat/1 -> mpc_pu_d/7(psi_alpha_hat)  "psi_alpha_hat"
  psi_beta_pu_hat/1 -> mpc_pu_d/8(psi_beta_hat)  "psi_beta_hat"
  [udcd_pu_inv_mod1] -> mpc_pu_d/1(vdc)
  Bus Creator1/1 -> ialpha/beta_tracking/1
  Bus Creator2/1 -> ialpha/beta_tracking/2
  mpc_pu_d/1(ualpha) -> Gain7/1
  mpc_pu_d/2(ubeta) -> Gain1/1
  Bus Creator/1 -> cmd_gates/1
  mpc_pu_d/3(cmg_g1) -> Bus Creator/1  "gate_cmd_Q1"
  mpc_pu_d/8(cmg_g6) -> Bus Creator/6  "gate_cmd_Q6"
  mpc_pu_d/7(cmg_g5) -> Bus Creator/5  "gate_cmd_Q5"
  mpc_pu_d/6(cmg_g4) -> Bus Creator/4  "gate_cmd_Q4"
  mpc_pu_d/5(cmg_g3) -> Bus Creator/3  "gate_cmd_Q3"
  mpc_pu_d/4(cmg_g2) -> Bus Creator/2  "gate_cmd_Q2"
  Gain7/1 -> Unit Delay/1
  Gain1/1 -> Unit Delay1/1
  Unit Delay/1 -> ualpha/1
  Unit Delay1/1 -> ubeta/1
  Constant1/1 -> mpc_pu_d/9(u_scale)
  Constant2/1 -> mpc_pu_d/10(L_norm)
  Constant3/1 -> mpc_pu_d/11(omega_bez)
  Constant4/1 -> mpc_pu_d/12(R_norm)
  Constant5/1 -> mpc_pu_d/13(k_kalman)
  Constant6/1 -> mpc_pu_d/14(k_sw)
  Constant7/1 -> mpc_pu_d/15(ts_inv)

== system mpc_psm/inv_psm_mod1/inverter_ctrl/inverter_control/is inv quantizzation and one step delay/is inv quantizzation and one step delay ==
  is_u_pu : Inport
  is_v_pu : Inport  Port=2
  is_w_pu : Inport  Port=3
  Gain3 : Gain  Gain=-1
  Gain4 : Gain  Gain=-1
  Gain5 : Gain  Gain=-1
  Quantizer : Quantizer  QuantizationInterval=param.meas.adc_quantization
  Quantizer1 : Quantizer  QuantizationInterval=param.meas.adc_quantization
  Quantizer2 : Quantizer  QuantizationInterval=param.meas.adc_quantization
  Unit Delay : UnitDelay  SampleTime=-1
  Unit Delay1 : UnitDelay  SampleTime=-1
  Unit Delay2 : UnitDelay  SampleTime=-1
  Zero-Order Hold : ZeroOrderHold  SampleTime=-1
  Zero-Order Hold1 : ZeroOrderHold  SampleTime=-1
  Zero-Order Hold2 : ZeroOrderHold  SampleTime=-1
  isd_u_pu : Outport
  isd_v_pu : Outport  Port=2
  isd_w_pu : Outport  Port=3
  wires:
  Unit Delay/1 -> Gain3/1
  Unit Delay1/1 -> Gain4/1
  Unit Delay2/1 -> Gain5/1
  Quantizer/1 -> Unit Delay/1
  Quantizer1/1 -> Unit Delay1/1
  Quantizer2/1 -> Unit Delay2/1
  is_u_pu/1 -> Zero-Order Hold/1
  is_v_pu/1 -> Zero-Order Hold1/1
  is_w_pu/1 -> Zero-Order Hold2/1
  Gain3/1 -> isd_u_pu/1
  Gain4/1 -> isd_v_pu/1
  Gain5/1 -> isd_w_pu/1
  Zero-Order Hold/1 -> Quantizer/1
  Zero-Order Hold1/1 -> Quantizer1/1
  Zero-Order Hold2/1 -> Quantizer2/1

== system mpc_psm/inv_psm_mod1/inverter_ctrl/inverter_control/omega_pu/flt ==
  input : Inport
  Gain3 : Gain  Gain=param.ctrl.filters.inv.g1_1Hz
  Gain6 : Gain  Gain=param.ctrl.filters.inv.g0_1Hz
  Sum : Sum  Inputs=|++
  Unit Delay1 : UnitDelay  SampleTime=-1
  output : Outport  VectorParamsAs1DForOutWhenUnconnected=off
  wires:
  Gain6/1 -> Sum/1
  input/1 -> Gain6/1
  Unit Delay1/1 -> Gain3/1
  Gain3/1 -> Sum/2
  Sum/1 -> Unit Delay1/1, output/1

== system mpc_psm/inv_psm_mod1/inverter_ctrl/inverter_control/phase_compensation_1/alignment_ctrl ==
  local_time : Inport
  master_time : Inport  Port=2
  Constant : Constant  Value=0
  Gain : Gain  Gain=-1
  Sum : Sum  Inputs=|+-
  pi : Subsystem  mask{kp=0 %param.ctrl.kp_align, ki=0 %param.ctrl.ki_align, lim_up=param.ctrl.lim_up_align, lim_down=param.ctrl.lim_down_align}
      mask prompts: ki "ki*ts"
      mask Display:
      | disp('pi()');
      | port_label('input', 1, 'u_ref');
      | port_label('input', 2, 'u');
      | port_label('output', 1, 'y');
  dp : Outport
  wires:
  master_time/1 -> Sum/1
  Sum/1 -> Gain/1
  Constant/1 -> pi/1(u_ref)
  local_time/1 -> Sum/2
  Gain/1 -> pi/2(u)
  pi/1(y) -> dp/1

== system mpc_psm/inv_psm_mod1/inverter_ctrl/inverter_control/speed_reference_generator/flt ==
  input : Inport
  Gain3 : Gain  Gain=param.ctrl.filters.inv.g1_1Hz
  Gain6 : Gain  Gain=param.ctrl.filters.inv.g0_1Hz
  Sum : Sum  Inputs=|++
  Unit Delay1 : UnitDelay  SampleTime=-1
  output : Outport  VectorParamsAs1DForOutWhenUnconnected=off
  wires:
  Gain6/1 -> Sum/1
  input/1 -> Gain6/1
  Unit Delay1/1 -> Gain3/1
  Gain3/1 -> Sum/2
  Sum/1 -> Unit Delay1/1, output/1

== system mpc_psm/inv_psm_mod1/inverter_ctrl/inverter_control/inner_ctrl/bemf_observer1/EKF_bemf_observer ==
  ialpha_pu : Inport
  ibeta_pu : Inport  Port=2
  ualpha_pu : Inport  Port=3
  ubeta_pu : Inport  Port=4
  udc_pu : Inport  Port=5
  EKF Observer simulink/Ccaller mod1 : Scope  NumInputPorts=2
      settings: ActiveDisplayYMinimum=-3.9268483156565956  ActiveDisplayYMaximum=3.9269848822951774
  Gain : Gain  Gain=param.psm.u_psm_scale_ekf
  Gain1 : Gain  Gain=param.psm.u_psm_scale_ekf
  Mux{,1..3} (4 alike) : Mux  Inputs=2
  Terminator : Terminator
  extended_kalman_observer : Subsystem
  phase_elec_ekf_hat : Outport
  omega_elec_ekf_hat : Outport  Port=2
  tag scope: psi_r_alpha_hat_mod1=scoped, psi_r_beta_hat_mod1=scoped
  wires:
  ialpha_pu/1 -> Mux2/1
  ibeta_pu/1 -> Mux2/2
  Mux/1 -> EKF Observer simulink/Ccaller mod1/1
  Mux1/1 -> EKF Observer simulink/Ccaller mod1/2
  extended_kalman_observer/3(phase_elec_ekf_hat) -> phase_elec_ekf_hat/1, Mux1/1  "phase_elec_ekf_hat"
  extended_kalman_observer/4(omega_elec_ekf_hat) -> omega_elec_ekf_hat/1, Mux/1  "omega_elec_ekf_hat"
  [omegad_pu_psm] -> Mux/2  "omega_pu_psm_encoder"
  [phased_psm] -> Mux1/2  "phase_psm_encoder"
  udc_pu/1 -> Terminator/1
  extended_kalman_observer/1(psi_alpha_ekf_hat) -> [psi_r_alpha_hat_mod1]
  extended_kalman_observer/2(psi_beta_ekf_hat) -> [psi_r_beta_hat_mod1]
  Mux2/1 -> extended_kalman_observer/2(ialphabeta)
  Mux3/1 -> extended_kalman_observer/1(ualphabeta)
  Gain/1 -> Mux3/1
  Gain1/1 -> Mux3/2
  ualpha_pu/1 -> Gain/1
  ubeta_pu/1 -> Gain1/1

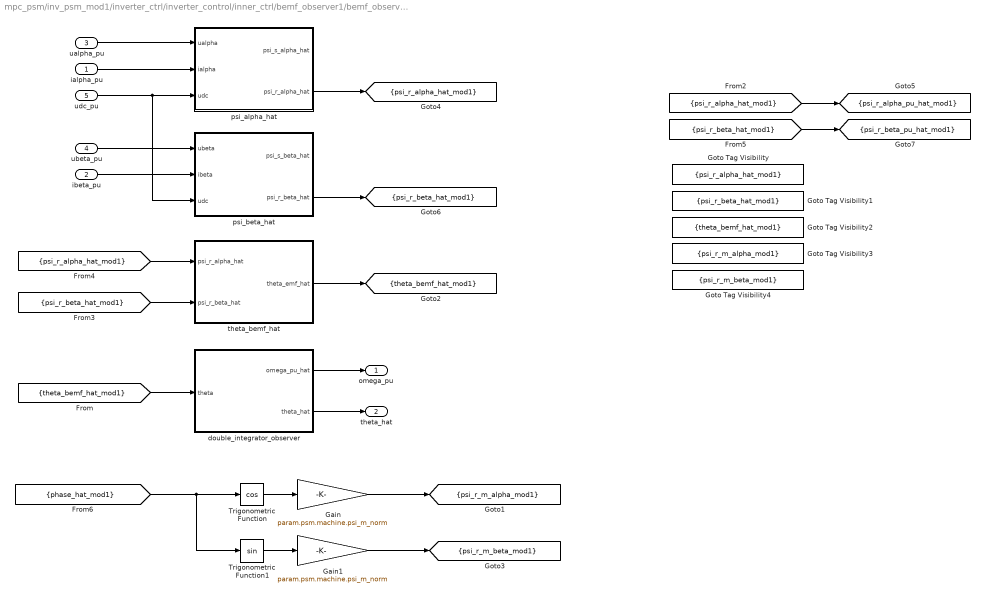
== system mpc_psm/inv_psm_mod1/inverter_ctrl/inverter_control/inner_ctrl/bemf_observer1/bemf_observer ==
  ialpha_pu : Inport
  ibeta_pu : Inport  Port=2
  ualpha_pu : Inport  Port=3
  ubeta_pu : Inport  Port=4
  udc_pu : Inport  Port=5
  Gain : Gain  Gain=param.psm.machine.psi_m_norm
  Gain1 : Gain  Gain=param.psm.machine.psi_m_norm
  Goto Tag Visibility : GotoTagVisibility  GotoTag=psi_r_alpha_hat_mod1
  Goto Tag Visibility1 : GotoTagVisibility  GotoTag=psi_r_beta_hat_mod1
  Goto Tag Visibility2 : GotoTagVisibility  GotoTag=theta_bemf_hat_mod1
  Goto Tag Visibility3 : GotoTagVisibility  GotoTag=psi_r_m_alpha_mod1
  Goto Tag Visibility4 : GotoTagVisibility  GotoTag=psi_r_m_beta_mod1
  Trigonometric Function : Trigonometry  Operator=cos
  Trigonometric Function1 : Trigonometry
  double_integrator_observer : Subsystem
  psi_alpha_hat : Subsystem
  psi_beta_hat : Subsystem
  theta_bemf_hat : Subsystem
  omega_pu : Outport
  theta_hat : Outport  Port=2
  tag scope: psi_r_alpha_hat_mod1=scoped, psi_r_alpha_pu_hat_mod1=scoped, psi_r_beta_hat_mod1=scoped, psi_r_beta_pu_hat_mod1=scoped, psi_r_m_alpha_mod1=scoped, psi_r_m_beta_mod1=scoped, theta_bemf_hat_mod1=scoped
  wires:
  Trigonometric Function/1 -> Gain/1
  Trigonometric Function1/1 -> Gain1/1
  ialpha_pu/1 -> psi_alpha_hat/2(ialpha)
  ibeta_pu/1 -> psi_beta_hat/2(ibeta)
  psi_alpha_hat/2(psi_r_alpha_hat) -> [psi_r_alpha_hat_mod1]
  psi_beta_hat/2(psi_r_beta_hat) -> [psi_r_beta_hat_mod1]
  [psi_r_alpha_hat_mod1] -> theta_bemf_hat/1(psi_r_alpha_hat)
  [psi_r_beta_hat_mod1] -> theta_bemf_hat/2(psi_r_beta_hat)
  ualpha_pu/1 -> psi_alpha_hat/1(ualpha)
  ubeta_pu/1 -> psi_beta_hat/1(ubeta)
  [phase_hat_mod1] -> Trigonometric Function/1, Trigonometric Function1/1
  Gain/1 -> [psi_r_m_alpha_mod1]
  Gain1/1 -> [psi_r_m_beta_mod1]
  theta_bemf_hat/1(theta_emf_hat) -> [theta_bemf_hat_mod1]
  [theta_bemf_hat_mod1] -> double_integrator_observer/1(theta)
  double_integrator_observer/1(omega_pu_hat) -> omega_pu/1
  double_integrator_observer/2(theta_hat) -> theta_hat/1
  [psi_r_alpha_hat_mod1] -> [psi_r_alpha_pu_hat_mod1]
  [psi_r_beta_hat_mod1] -> [psi_r_beta_pu_hat_mod1]
  udc_pu/1 -> psi_alpha_hat/3(udc), psi_beta_hat/3(udc)

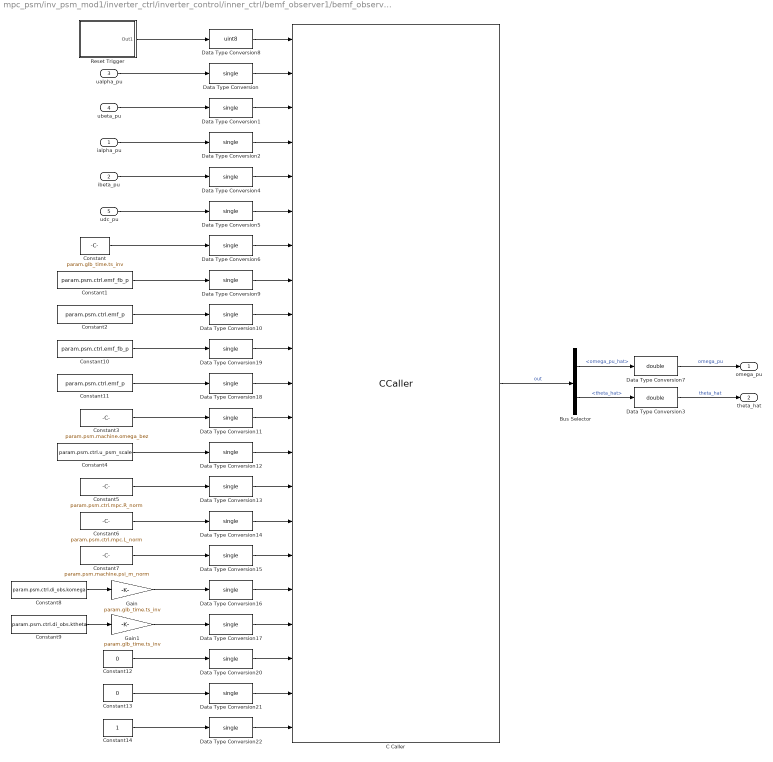
== system mpc_psm/inv_psm_mod1/inverter_ctrl/inverter_control/inner_ctrl/bemf_observer1/bemf_observer_ccaller ==
  ialpha_pu : Inport
  ibeta_pu : Inport  Port=2
  ualpha_pu : Inport  Port=3
  ubeta_pu : Inport  Port=4
  udc_pu : Inport  Port=5
  Bus Selector : BusSelector  OutputSignals=omega_pu_hat,theta_hat
  C Caller : CCaller  FunctionName=bemf_obsv_process_simulink  PortSpecificationStruct="%)30     .    N\"8   8    (     @         %    \"    !8    !     0         %  0 \"0    $    _    07)G3F%M90  4&]R=$YA;64 4V-O<&4     26YD97@     5'EP90      4VEZ90      27-';&]B86P   X    P    !@    @    $          4    (     0    ,    !         !   P!O=70 #@   #     &    \"     0         !0    @    !     P    $         $  # &]U=  .    .     8    (    !          %    \"     $    &     0         0  ...(+12985 chars)"
  Constant : Constant  Value=param.glb_time.ts_inv
  Constant1 : Constant  Value=param.psm.ctrl.emf_fb_p
  Constant10 : Constant  Value=param.psm.ctrl.emf_fb_p
  Constant11 : Constant  Value=param.psm.ctrl.emf_p
  Constant12 : Constant  Value=0
  Constant13 : Constant  Value=0
  Constant14 : Constant
  Constant2 : Constant  Value=param.psm.ctrl.emf_p
  Constant3 : Constant  Value=param.psm.machine.omega_bez
  Constant4 : Constant  Value=param.psm.ctrl.u_psm_scale
  Constant5 : Constant  Value=param.psm.ctrl.mpc.R_norm
  Constant6 : Constant  Value=param.psm.ctrl.mpc.L_norm
  Constant7 : Constant  Value=param.psm.machine.psi_m_norm
  Constant8 : Constant  Value=param.psm.ctrl.di_obs.komega
  Constant9 : Constant  Value=param.psm.ctrl.di_obs.ktheta
  Data Type Conversion{,1..2,4..6,9..22} (20 alike) : DataTypeConversion  OutDataTypeStr=single  SaturateOnIntegerOverflow=off  RndMeth=Floor
  Data Type Conversion3 : DataTypeConversion  OutDataTypeStr=double  SaturateOnIntegerOverflow=off  RndMeth=Floor
  Data Type Conversion7 : DataTypeConversion  OutDataTypeStr=double  SaturateOnIntegerOverflow=off  RndMeth=Floor
  Data Type Conversion8 : DataTypeConversion  OutDataTypeStr=uint8  SaturateOnIntegerOverflow=off  RndMeth=Floor
  Gain : Gain  Gain=param.glb_time.ts_inv
  Gain1 : Gain  Gain=param.glb_time.ts_inv
  Reset Trigger : Subsystem
  omega_pu : Outport
  theta_hat : Outport  Port=2
  wires:
  Data Type Conversion5/1 -> C Caller/6
  Data Type Conversion/1 -> C Caller/2
  C Caller/1 -> Bus Selector/1  "out"
  Data Type Conversion1/1 -> C Caller/3
  Data Type Conversion4/1 -> C Caller/5
  Data Type Conversion2/1 -> C Caller/4
  Data Type Conversion6/1 -> C Caller/7
  Bus Selector/2 -> Data Type Conversion3/1  "<theta_hat>"
  Bus Selector/1 -> Data Type Conversion7/1  "<omega_pu_hat>"
  Data Type Conversion7/1 -> omega_pu/1  "omega_pu"
  Data Type Conversion3/1 -> theta_hat/1  "theta_hat"
  Data Type Conversion8/1 -> C Caller/1
  Data Type Conversion9/1 -> C Caller/8
  Data Type Conversion10/1 -> C Caller/9
  Data Type Conversion19/1 -> C Caller/10
  Data Type Conversion18/1 -> C Caller/11
  Data Type Conversion11/1 -> C Caller/12
  Data Type Conversion12/1 -> C Caller/13
  Data Type Conversion13/1 -> C Caller/14
  Data Type Conversion14/1 -> C Caller/15
  Data Type Conversion15/1 -> C Caller/16
  Data Type Conversion16/1 -> C Caller/17
  Data Type Conversion17/1 -> C Caller/18
  Data Type Conversion20/1 -> C Caller/19
  Data Type Conversion21/1 -> C Caller/20
  Data Type Conversion22/1 -> C Caller/21
  Constant14/1 -> Data Type Conversion22/1
  Constant13/1 -> Data Type Conversion21/1
  Constant12/1 -> Data Type Conversion20/1
  Constant9/1 -> Gain1/1
  Constant8/1 -> Gain/1
  Constant7/1 -> Data Type Conversion15/1
  Constant6/1 -> Data Type Conversion14/1
  Constant5/1 -> Data Type Conversion13/1
  Constant4/1 -> Data Type Conversion12/1
  Constant3/1 -> Data Type Conversion11/1
  Constant11/1 -> Data Type Conversion18/1
  Constant10/1 -> Data Type Conversion19/1
  Constant2/1 -> Data Type Conversion10/1
  Constant1/1 -> Data Type Conversion9/1
  Constant/1 -> Data Type Conversion6/1
  ibeta_pu/1 -> Data Type Conversion4/1
  ialpha_pu/1 -> Data Type Conversion2/1
  ubeta_pu/1 -> Data Type Conversion1/1
  ualpha_pu/1 -> Data Type Conversion/1
  Reset Trigger/1(Out1) -> Data Type Conversion8/1
  udc_pu/1 -> Data Type Conversion5/1
  Gain/1 -> Data Type Conversion16/1
  Gain1/1 -> Data Type Conversion17/1
